simulink model "HarnessModel_BEVController"  (R2026a)
settings: Solver=daessc  StopTime=2000  AbsTol=1e-3
PreLoadFcn:
  | setupHarness_BEVController
undefined symbols (not defined in the file or in its folder): VehicleSpeedInput
libraries: simulink x1
settings Model: Creator=isaacito  LastModifiedBy=isaacito
settings SimscapeCC: SimscapeNominalValues="[{\"value\":\"1\",\"unit\":\"A\"},{\"value\":\"1\",\"unit\":\"bar\"},{\"value\":\"1\",\"unit\":\"cm^2\"},{\"value\":\"1\",\"unit\":\"cm^3/s\"},{\"value\":\"1\",\"unit\":\"kJ/kg\"},{\"value\":\"1\",\"unit\":\"kW\"},{\"value\":\"1\",\"unit\":\"l\"},{\"value\":\"1\",\"unit\":\"N\"},{\"value\":\"1\",\"unit\":\"N*m\"},{\"value\":\"1\",\"unit\":\"V\"}]"  SimscapeLogSimulationStatistics=on  SimscapeLogLimitData=off  SimscapeLogDataHistory=5000.0

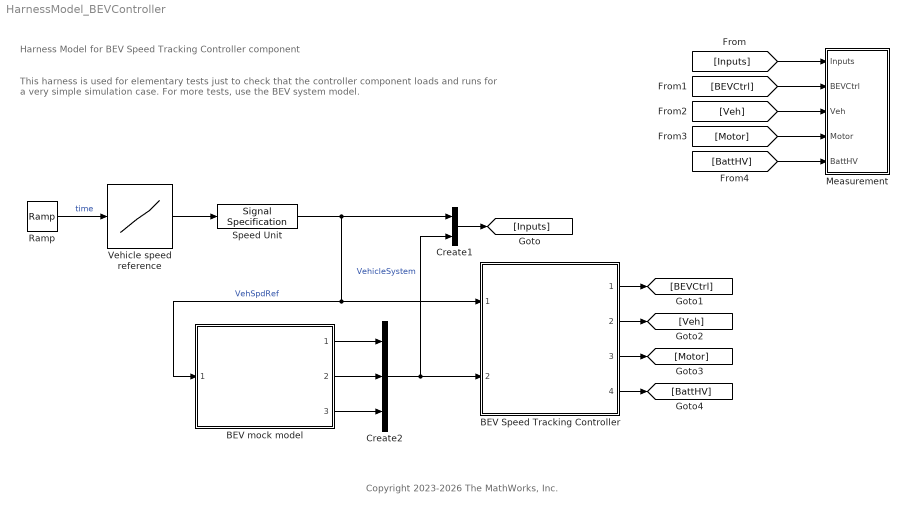
== system HarnessModel_BEVController ==
  note: This harness is used for elementary tests
      | just to check that the controller component loads and runs
      | for a very simple simulation case.
      | For more tests, use the BEV system model.
  note: Harness Model for BEV Speed Tracking Controller component
  note: Copyright 2023-2026 The MathWorks, Inc.
  BEV Speed Tracking Controller : Subsystem  ReferencedSubsystem=BEVController_Basic_refsub
      settings: OpenFcn=|
      | % Look under mask:
      | open_system(gcb, "force")
  BEV mock model : Subsystem  ReferencedSubsystem=BEV_MockModel_refsub
      settings: OpenFcn="open_system(gcb, \"force\")"
  Create1 : BusCreator  Inputs=2
  Create2 : BusCreator  Inputs=3
  Measurement : Subsystem
  Ramp : simulink/Sources/Ramp  slope=1  start=0  InitialOutput=0
      settings: AttributesFormatString=|
      | Slope: %<slope>
      | Start time: %<start>
      | Initial output: %<InitialOutput>
  Speed Unit : SignalSpecification  Unit=km/h
  Vehicle speed reference : Lookup_n-D  NumberOfTableDimensions=1  BreakpointsForDimension1="VehicleSpeedInput.Time.value(\"s\")"  Table="VehicleSpeedInput.Speed.value(\"km/hr\")"  InterpMethod=Akima spline  InternalRulePriority=Speed  RndMeth=Simplest
  wires:
  BEV Speed Tracking Controller/1 -> [BEVCtrl]
  BEV Speed Tracking Controller/2 -> [Veh]
  BEV Speed Tracking Controller/3 -> [Motor]
  BEV Speed Tracking Controller/4 -> [BattHV]
  [Inputs] -> Measurement/1(Inputs)
  [BEVCtrl] -> Measurement/2(BEVCtrl)
  [Veh] -> Measurement/3(Veh)
  [Motor] -> Measurement/4(Motor)
  [BattHV] -> Measurement/5(BattHV)
  BEV mock model/2 -> Create2/2
  Create1/1 -> [Inputs]
  Vehicle speed reference/1 -> Speed Unit/1
  BEV mock model/3 -> Create2/3
  Create2/1 -> Create1/2, BEV Speed Tracking Controller/2  "VehicleSystem"
  Ramp/1 -> Vehicle speed reference/1  "time"
  BEV mock model/1 -> Create2/1
  Speed Unit/1 -> BEV mock model/1, BEV Speed Tracking Controller/1, Create1/1  "VehSpdRef"

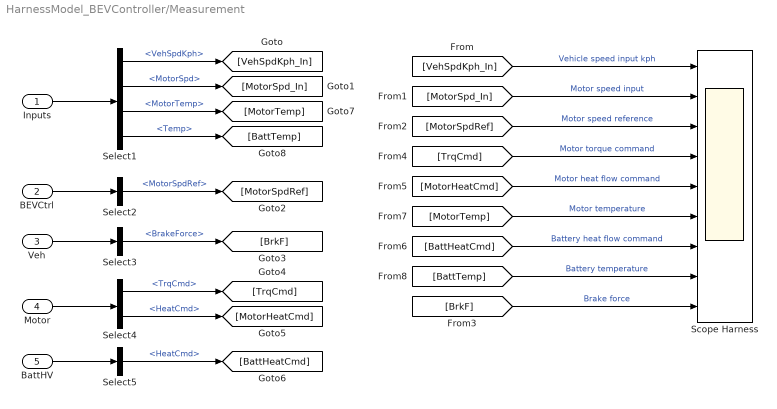
== system HarnessModel_BEVController/Measurement ==
  Inputs : Inport
  BEVCtrl : Inport  Port=2
  Veh : Inport  Port=3
  Motor : Inport  Port=4
  BattHV : Inport  Port=5
  Scope Harness : Scope  NumInputPorts=9
      settings: ActiveDisplayYMinimum=-12.501622080778102  ActiveDisplayYMaximum=112.51449532901584
  Select1 : BusSelector  OutputSignals=VehicleSystem.Vehicle.VehSpdKph,VehicleSystem.Motor.MotorSpd,VehicleSystem.Motor.MotorTemp,VehicleSystem.Battery.Temp
  Select2 : BusSelector  OutputSignals=MotorSpdRef
  Select3 : BusSelector  OutputSignals=BrakeForce
  Select4 : BusSelector  OutputSignals=TrqCmd,HeatCmd
  Select5 : BusSelector  OutputSignals=HeatCmd
  wires:
  Inputs/1 -> Select1/1
  Select1/1 -> [VehSpdKph_In]  "<VehSpdKph>"
  Select1/2 -> [MotorSpd_In]  "<MotorSpd>"
  BEVCtrl/1 -> Select2/1
  Select2/1 -> [MotorSpdRef]  "<MotorSpdRef>"
  Veh/1 -> Select3/1
  Select3/1 -> [BrkF]  "<BrakeForce>"
  Motor/1 -> Select4/1
  Select4/1 -> [TrqCmd]  "<TrqCmd>"
  Select4/2 -> [MotorHeatCmd]  "<HeatCmd>"
  BattHV/1 -> Select5/1
  Select5/1 -> [BattHeatCmd]  "<HeatCmd>"
  [VehSpdKph_In] -> Scope Harness/1  "Vehicle speed input kph"
  [MotorSpd_In] -> Scope Harness/2  "Motor speed input"
  [MotorSpdRef] -> Scope Harness/3  "Motor speed reference"
  Select1/3 -> [MotorTemp]  "<MotorTemp>"
  Select1/4 -> [BattTemp]  "<Temp>"
  [TrqCmd] -> Scope Harness/4  "Motor torque command"
  [MotorHeatCmd] -> Scope Harness/5  "Motor heat flow command"
  [MotorTemp] -> Scope Harness/6  "Motor temperature"
  [BattHeatCmd] -> Scope Harness/7  "Battery heat flow command"
  [BattTemp] -> Scope Harness/8  "Battery temperature"
  [BrkF] -> Scope Harness/9  "Brake force"
